simulink model "baseline_source"  (R2025a)
settings: Solver=daessc  StartTime=0.0  StopTime=25  MaxStep=5e-6  RelTol=1e-3
model workspace (MAT data in the model file):
  FocDiscrTime = 8.33333333333e-05
  Is_max = 420
  Ld = 0.00031
  Lq = 0.000305
  PolePairs = 11
  Psi = 0.1024
  Rs = 0.02
  VDC = 440
  compensate_dt = 0
  compensate_pwm = 0
  deltaLd = 0.2
  deltaLq = 0
  deltaPsi = 0
  deltaRs = 0
  mFW = 0.95
  mMaxCurrent = 0.99
  mMaxPWM = 0.99
  piBandwidth = 6000
libraries: fl_lib x18, nesl_utility x15, eeGeneralControl x9, mcbeeMathTransformLib x7, simulink x7, slpidlib x5, spsMeanLib x4, ee_lib x1, simulink_extras x1
(part 1 of 2)
settings Model: SimulationMode=rapid-accelerator  ExtModeTrigDuration=100  Creator=alexey  LastModifiedBy=alexey
settings SolverCC: ZeroCrossAlgorithm=Adaptive
settings OptimizationCC: DefaultParameterBehavior=Inlined  UseDivisionForNetSlopeComputation=on  GainParamInheritBuiltInType=on  UseFloatMulNetSlope=on  InlineInvariantSignals=on  ReuseModelBlockBuffer=off  EfficientFloat2IntCast=on  LifeSpan=1
settings DebuggingCC: MaskedZcDiagnostic=none  IgnoredZcDiagnostic=none
settings HardwareCC: ProdLongLongMode=on
settings SFSimCC: MATLABDynamicMemAlloc=off
settings RTWCC: GenerateReport=on  LaunchReport=on  GPUComputeCapability=3.5
settings CodeAppCC: ForceParamTrailComments=on
settings GRTTargetCC: RTWCAPISignals=on  RTWCAPIParams=on  CombineSignalStateStructs=on  MatFileLogging=off  SupportVariableSizeSignals=on

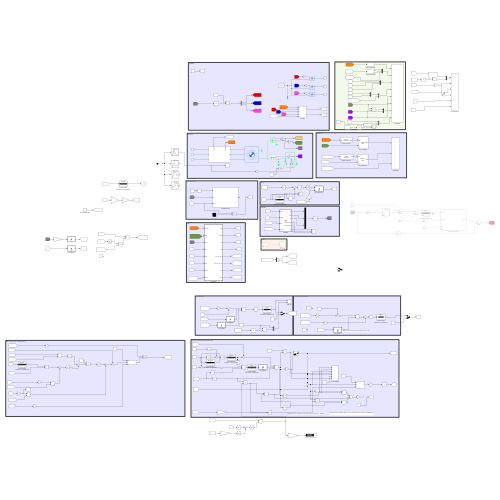
[thumbnail: Simulink's stored preview of the top-level diagram]
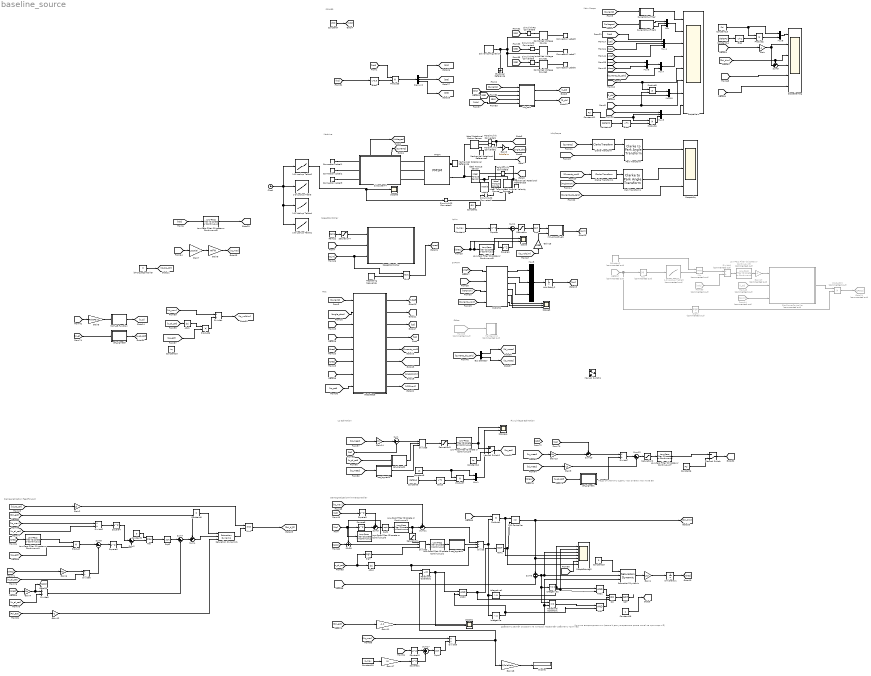
== system baseline_source ==
  note: Надо отключить оценку при омегах мех ниже 50
  note: Изучить вопрос динамики (роста U для ускоренного роста тока) на триммер и ff/
  note: Добавить расчёт скорости на которой перестаёт работать триммер
  note: Lq estimation
  note: Demagnetization FeedForward
  note: FluxLinkage Estimation
  note: Other
  note: SVPWM
  note: FOC
  note: IqLim
  note: DemagnetizationTrimmerController
  note: IdIqScope
  note: SpeedController
  note: Machine
  note: Main Scope
  note: POWER
  1-D Lookup Table : Lookup_n-D  NumberOfTableDimensions=1  BreakpointsForDimension1=[0 0.4 0.45 0.55 0.87 1 1.5 1.6 1.7]  Table=[0 308 308 104 104 120 120 220 220]  InternalRulePriority=Speed  RndMeth=Simplest
  1-D Lookup Table1 : Lookup_n-D  NumberOfTableDimensions=1  BreakpointsForDimension1=[0 0.2 0.4 4 4.2 8 8.2 9.0]  Table=[0 0 204 204 408 408 204 204]  InternalRulePriority=Speed  RndMeth=Simplest
  1-D Lookup Table2 : Lookup_n-D  NumberOfTableDimensions=1  BreakpointsForDimension1=[0 0.3 1 1.3 2 2.3 3 3.3 4 4.3 5 5.3 6 6.3 7 14 24 ]  Table=[0 104 104 208 208 312 312 416 416 520 520 624 624 738 738 156 21]  InternalRulePriority=Speed  RndMeth=Simplest
  1-D Lookup Table3 : Lookup_n-D  Commented=on  NumberOfTableDimensions=1  BreakpointsForDimension1=[0 550 600 1000 1925 2350 2400 2450]*0.1047  Table=[0 0 30000 48500 48500 22000 0 0]  InternalRulePriority=Speed  RndMeth=Simplest
  1-D Lookup Table4 : Lookup_n-D  NumberOfTableDimensions=1  BreakpointsForDimension1=[0 0.4 1.0 1.2 1.8]  Table=[0 408 408 204 204]  InternalRulePriority=Speed  RndMeth=Simplest
  AND : Logic  IconShape=distinctive  AllPortsSameDT=off  OutDataTypeStr=boolean
  AND1 : Logic  IconShape=distinctive  AllPortsSameDT=off  OutDataTypeStr=boolean
  AND2 : Logic  IconShape=distinctive  AllPortsSameDT=off  OutDataTypeStr=boolean
  Abs : Abs  Commented=on  SaturateOnIntegerOverflow=off
  Abs1 : Abs  SaturateOnIntegerOverflow=off
  Abs4 : Abs  SaturateOnIntegerOverflow=off
  Bias : Bias  Bias=1  SaturateOnIntegerOverflow=off
  Bias1 : Bias  Bias=1  SaturateOnIntegerOverflow=off
  Bias2 : Bias  Bias=-0.5  SaturateOnIntegerOverflow=off
  Bias3 : Bias  Bias=1  SaturateOnIntegerOverflow=off
  Bus Selector : BusSelector  OutputSignals=Id,Iq
  Clarke Transform : mcbeeMathTransformLib/Clarke Transform  VariantControl=Variant2  PowerInvariant=off  UseWithEmbedded=on  PhaseInput=Three inputs
      settings: LibrarySourceBlock=mcbcontrolslib/Clarke Transform
  Clarke Transform1 : mcbeeMathTransformLib/Clarke Transform  VariantControl=Variant2  PowerInvariant=off  UseWithEmbedded=on  PhaseInput=Three inputs
      settings: LibrarySourceBlock=mcbcontrolslib/Clarke Transform
  Clock : Clock
  Connection Label1 : ConnectionLabel  Label=A
  Connection Label2 : ConnectionLabel  Label=B
  Connection Label6 : ConnectionLabel  Label=C
  Connection Label7 : ConnectionLabel  Label=B
  Connection Label8 : ConnectionLabel  Label=A
  Connection Label9 : ConnectionLabel  Label=C
  Constant : Constant  Value=Is_max
  Constant1 : Constant  Value=-50
  Constant10 : Constant  Value=Lq
  Constant11 : Constant  Value=Psi
  Constant12 : Constant  Value=Lq  SampleTime=FocDiscrTime
  Constant13 : Constant  Value=Psi
  Constant14 : Constant  Value=deltaPsi
  Constant15 : Constant  Value=0
  Constant16 : Constant
  Constant18 : Constant  Value=Is_max
  Constant2 : Constant  Value=0
  Constant3 : Constant  Value=0
  Constant4 : Constant  Value=deltaPsi
  Constant5 : Constant  Commented=on  Value=48500
  Constant6 : Constant  Value=Psi  SampleTime=FocDiscrTime
  Constant7 : Constant  Value=VDC
  Constant8 : Constant  Value=Lq
  Constant9 : Constant  Value=deltaLq
  Controlled Voltage Source : fl_lib/Electrical/Electrical Sources/Controlled Voltage Source
  Controlled Voltage Source1 : fl_lib/Electrical/Electrical Sources/Controlled Voltage Source
  Controlled Voltage Source2 : fl_lib/Electrical/Electrical Sources/Controlled Voltage Source
  CurrentsMuxFilter : Subsystem
  CurrentsMuxFilter1 : Subsystem
  Demux2 : Demux  Outputs=3
  Display : Display
  Divide : Product  Inputs=*//
  Divide1 : Product  Commented=on  Inputs=*/
  Divide{2,4..7,9} (6 alike) : Product  Inputs=*/
  Divide3 : Product  Inputs=/**
  Divide8 : Product  Inputs=*//
  Electrical Reference : fl_lib/Electrical/Electrical Elements/Electrical Reference
  From38 : From  Commented=on  GotoTag=angle_mech
  From44 : From  Commented=on  GotoTag=IqLim
  From45 : From  Commented=on  GotoTag=I_dc
  From47 : From  Commented=on  GotoTag=speed
  From50 : From  Commented=on  GotoTag=Vdc
  Gain : Gain  Gain=-1
  Gain1 : Gain  Gain=1/Ld
  Gain10 : Gain  Commented=on  Gain=-1
  Gain11 : Gain  Gain=-1.2
  Gain12 : Gain  Gain=-1
  Gain{4,6,13..14} (4 alike) : Gain  Gain=Rs
  Gain15 : Gain  Gain=0.95
  Gain17 : Gain  Gain=Lq
  Gain18 : Gain  Gain=1/PolePairs
  Gain2 : Gain  Gain=Ld
  Gain3 : Gain  Gain=PolePairs
  Gain5 : Gain  Gain=PolePairs
  Gain7 : Gain  Gain=1/sqrt(3)
  Gain8 : Gain  Gain=mFW
  Gain9 : Gain  Gain=Ld
  GenPowerController : Subsystem  Commented=on
  Goto24 : Goto  Commented=on  GotoTag=IqReq1
  HallSensors : Subsystem  Commented=on
  Idc_calc : Subsystem
  Ideal Angular Velocity Source : fl_lib/Mechanical/Mechanical Sources/Ideal Angular Velocity Source
  Ideal Rotational Motion Sensor : fl_lib/Mechanical/Mechanical Sensors/Ideal Rotational Motion Sensor  reference=foundation.enum.MeasurementReference.difference  acceleration_port=false  velocity_port=true  position_port=true  wrap_angle=false  offset=0 rad
  Ideal Torque Sensor : fl_lib/Mechanical/Mechanical Sensors/Ideal Torque Sensor
  Ideal Torque Source : fl_lib/Mechanical/Mechanical Sources/Ideal Torque Source
  Inertia : fl_lib/Mechanical/Rotational Elements/Inertia  inertia=0.1 kg*m^2  num_ports=foundation.enum.numPorts2.one  w_specify=off  w_priority=High  w=0 rad/s  w_nominal_specify=off  w_nominal_value=1  w_nominal_unit=rad/s  t_specify=off  t_priority=None  t=0 N*m  t_nominal_specify=off  t_nominal_value=1  t_nominal_unit=N*m
  IsNegative : simulink/Logic and Bit Operations/Compare To Zero  relop=<  OutDataTypeStr=uint8
      settings: LibrarySourceBlock=|
      | simulink/Quick Insert/Logic and Bit
      | Operations/IsNegative
  IsNegative1 : simulink/Logic and Bit Operations/Compare To Zero  relop=>  OutDataTypeStr=uint8
      settings: LibrarySourceBlock=|
      | simulink/Quick Insert/Logic and Bit
      | Operations/IsNegative
  IsNegative2 : simulink/Logic and Bit Operations/Compare To Zero  relop=>=  OutDataTypeStr=uint8
      settings: LibrarySourceBlock=|
      | simulink/Quick Insert/Logic and Bit
      | Operations/IsNegative
  Low-Pass Filter (Discrete or Continuous)1 : eeGeneralControl/Low-Pass Filter (Discrete or Continuous)  K=1  T=FocDiscrTime*10  B=inf  A=-inf  init_option=Specify as parameter  x0=0  Ts=FocDiscrTime
  Low-Pass Filter (Discrete or Continuous)2 : eeGeneralControl/Low-Pass Filter (Discrete or Continuous)  K=1  T=FocDiscrTime*10  B=inf  A=-inf  init_option=Specify as parameter  x0=0  Ts=FocDiscrTime
  Low-Pass Filter (Discrete or Continuous)3 : eeGeneralControl/Low-Pass Filter (Discrete or Continuous)  Commented=on  K=1  T=FocDiscrTime*20  B=1.4*Psi  A=-inf  init_option=Specify as parameter  x0=Psi  Ts=FocDiscrTime
  Low-Pass Filter (Discrete or Continuous)4 : eeGeneralControl/Low-Pass Filter (Discrete or Continuous)  K=1  T=FocDiscrTime*10  B=inf  A=-inf  init_option=Inherited from block input  x0=0  Ts=FocDiscrTime
  Low-Pass Filter (Discrete or Continuous)5 : eeGeneralControl/Low-Pass Filter (Discrete or Continuous)  K=1  T=FocDiscrTime*20  B=inf  A=-inf  init_option=Specify as parameter  x0=VDC  Ts=FocDiscrTime
  Low-Pass Filter (Discrete or Continuous)6 : eeGeneralControl/Low-Pass Filter (Discrete or Continuous)  K=1  T=FocDiscrTime*10  B=inf  A=-inf  init_option=Specify as parameter  x0=0  Ts=FocDiscrTime
  Low-Pass Filter (Discrete or Continuous)7 : eeGeneralControl/Low-Pass Filter (Discrete or Continuous)  K=1  T=FocDiscrTime*20000  B=1.4*Psi  A=0.6*Psi  init_option=Specify as parameter  x0=Psi  Ts=FocDiscrTime
  Low-Pass Filter (Discrete or Continuous)8 : eeGeneralControl/Low-Pass Filter (Discrete or Continuous)  K=1  T=FocDiscrTime*100  B=inf  A=-inf  init_option=Specify as parameter  x0=0  Ts=FocDiscrTime
  Low-Pass Filter (Discrete or Continuous)9 : eeGeneralControl/Low-Pass Filter (Discrete or Continuous)  K=1  T=FocDiscrTime*200  B=inf  A=-inf  init_option=Specify as parameter  x0=Lq  Ts=FocDiscrTime
  MATLAB Function : MATLAB Function  TreatAsAtomicUnit=on
  Manual Switch : ManualSwitch  CurrentSetting=0
  Manual Switch1 : ManualSwitch
  Manual Switch2 : ManualSwitch  CurrentSetting=0
  Max : MinMax  Function=max  Inputs=2
  Mechanical Rotational Reference : fl_lib/Mechanical/Rotational Elements/Mechanical Rotational Reference
  Mechanical Rotational Reference2 : fl_lib/Mechanical/Rotational Elements/Mechanical Rotational Reference
  Mechanical Rotational Reference3 : fl_lib/Mechanical/Rotational Elements/Mechanical Rotational Reference
  Min : MinMax  Commented=on  Inputs=2
  Min1 : MinMax  Inputs=2
  Min3 : MinMax  Inputs=2
  Min_smooth_ab : MATLAB Function  TreatAsAtomicUnit=on
  Mux{,3..5} (4 alike) : Mux  Inputs=3
  Mux{1,6..8,10} (5 alike) : Mux  Inputs=2
  NOT : Logic  Operator=NOT  IconShape=distinctive  AllPortsSameDT=off  OutDataTypeStr=boolean
  NOT1 : Logic  Operator=NOT  IconShape=distinctive  AllPortsSameDT=off  OutDataTypeStr=boolean
  OR : Logic  Operator=OR  Inputs=3  IconShape=distinctive  AllPortsSameDT=off  OutDataTypeStr=boolean
  PID Controller : slpidlib/PID Controller  Controller=I  Form=Parallel  TimeDomain=Discrete-time  UseExternalTs=off  SampleTime=FocDiscrTime*1  IntegratorMethod=Forward Euler  FilterMethod=Forward Euler  ControllerParametersSource=internal  P=0  I=45  UseKiTs=off  D=0  UseExternalDerivativeSource=off  N=100  UseFilter=on  TunerSelectOption=Transfer Function Based (PID Tuner App)  InitialConditionSource=internal  InitialConditionForIntegrator=0  InitialConditionForFilter=0  DifferentiatorICPrevScaledInput=0  ExternalReset=either  TrackingMode=off  Kt=1  LimitOutput=on  SatLimitsSource=internal  UpperSaturationLimit=500*Ld  LowerSaturationLimit=-500*Ld  LinearizeAsGain=off  AntiWindupMode=clamping  Kb=1  LimitIntegrator=off  UpperIntegratorSaturationLimit=inf  LowerIntegratorSaturationLimit=-inf  RndMeth=Round  POutMin=[]  POutMax=[]  IOutMin=[]  IOutMax=[]  DOutMin=[]  DOutMax=[]  NOutMin=[]  NOutMax=[]  SumOutMin=[]  SumOutMax=[]  SaturationOutMin=[]  SaturationOutMax=[]  PParamMin=[]  PParamMax=[]  IParamMin=[]  IParamMax=[]  DParamMin=[]  DParamMax=[]  NParamMin=[]  NParamMax=[]  KbParamMin=[]  KbParamMax=[]  KtParamMin=[]  KtParamMax=[]  KbOutMin=[]  KbOutMax=[]  KtOutMin=[]  KtOutMax=[]  IntegratorOutMin=[]  IntegratorOutMax=[]  FilterOutMin=[]  FilterOutMax=[]  SumI1OutMin=[]  SumI1OutMax=[]  SumI2OutMin=[]  SumI2OutMax=[]  SumI3OutMin=[]  SumI3OutMax=[]  SumI4OutMin=[]  SumI4OutMax=[]  SumDOutMin=[]  SumDOutMax=[]  DifferentiatorOutMin=[]  DifferentiatorOutMax=[]  FilterDiffOutCoefMin=[]  FilterDiffOutCoefMax=[]  ReciprocalOutMin=[]  ReciprocalOutMax=[]  SumDenOutMin=[]  SumDenOutMax=[]  SumNumOutMin=[]  SumNumOutMax=[]  DivideOutMin=[]  DivideOutMax=[]  UdiffTsProdOutMin=[]  UdiffTsProdOutMax=[]  NTsProdOutMin=[]  NTsProdOutMax=[]  UintegralTsProdOutMin=[]  UintegralTsProdOutMax=[]  UngainTsProdOutMin=[]  UngainTsProdOutMax=[]  ClampingZeroOutDataTypeStr=Inherit: Inherit via back propagation  ClampingZeroOutMin=[]  ClampingZeroOutMax=[]  FilterDenConstantOutDataTypeStr=Inherit: Inherit via back propagation  FilterDenConstantOutMin=[]  FilterDenConstantOutMax=[]  PCopyOutDataTypeStr=Inherit: Inherit via back propagation  PCopyOutMin=[]  PCopyOutMax=[]  NCopyOutDataTypeStr=Inherit: Inherit via back propagation  NCopyOutMin=[]  NCopyOutMax=[]  IntegratorContinuousStateAttributes=''  IntegratorStateMustResolveToSignalObject=off  IntegratorRTWStateStorageClass=Auto  FilterContinuousStateAttributes=''  FilterStateMustResolveToSignalObject=off  FilterRTWStateStorageClass=Auto  ParallelPVariant=Disabled  IdealPVariant=Disabled  IVariant=InternalParameters  DVariant=Disabled  IntegratorVariant=Discrete  SatVariant=Enabled  AWVariant=DiscClampingParallel  PCopyVariant=Disabled  TRVariant=Disabled  FdbkBlocksVariant=Forward  IdealPFdbkVariant=Disabled  SatFdbkVariant=Disabled  DerivativeFilterVariant=Disabled  NVariant=Disabled  NCopyVariant=Disabled_SignalSpec  FilterICVariant=Disabled  IntegratorICVariant=InternalICs  ExternalResetVariant=ExternalReset  TRSumVariant=Passthrough  SumFdbkVariant=Disabled  SumVariant=Passthrough_I  TsampFilterVariant=InternalTs  TsampNgainVariant=Passthrough  TsampIntegralVariant=Disabled_SignalSpec  ExternalSaturationOutDataTypeStr=Inherit: Same as second input  DerivativeSourceVariant=Disabled  PreIntVariant=InternalPreInt
  PMSM : ee_lib/Electromechanical/Permanent Magnet/PMSM  port_option=ee.enum.threePhasePort.expanded  winding_type=ee.enum.electromech.statorconfiguration.wye  machine_param=ee.enum.pmsm.parameterization.constant  nPolePairs=PolePairs  pmflux_param=ee.enum.pmflux.fluxlinkage  pm_flux_linkage=Psi*(1+deltaPsi) Wb  torque_constant=0.074 N*m/A  back_emf_constant=0.06 V*s/rad  stator_param=ee.enum.statorparam.LdLqL0  Ld=Ld*(1+deltaLd) H  Lq=Lq*(1+deltaLq) H  idVec=[-200, 0, 200] A  iqVec=[-200, 0, 200] A  LdMatrix=0.0002 * ones(3, 3) H  LqMatrix=0.0002 * ones(3, 3) H  PmMatrix=0.1 * ones(3, 3) Wb  ktMatrix=0.18 * ones(3, 3) N*m/A  keMatrix=0.18 * ones(3, 3) V*s/rad  L0=1e-6 uH  Ls=0.0002 H  Lm=-0.00002 H  Ms=0.00002 H  Rs=Rs*(1+deltaRs) Ohm  zero_sequence=ee.enum.park.zerosequence.exclude  axes_param=ee.enum.rotorangle.daxis  loss_param=ee.enum.ironloss.none  losses_oc=[0, 0, 0] W  losses_sc=[0, 0, 0] W  f_losses=60 Hz  Isc_losses=95 A  J=0 kg*m^2  lam=0 N*m*s/rad  i_d_specify=on  i_d_priority=High  i_d=0 A  i_d_nominal_specify=off  i_d_nominal_value=1  i_d_nominal_unit=A  i_q_specify=on  i_q_priority=High  i_q=0 A  i_q_nominal_specify=off  i_q_nominal_value=1  i_q_nominal_unit=A  torque_specify=on  torque_priority=High  torque=0 N*m  torque_nominal_specify=off  torque_nominal_value=1  torque_nominal_unit=N*m  angular_velocity_specify=on  angular_velocity_priority=None  angular_velocity=7000 rpm  angular_velocity_nominal_specify=off  angular_velocity_nominal_value=1  angular_velocity_nominal_unit=rpm  angular_position_specify=on  angular_position_priority=High  angular_position=0 deg  angular_position_nominal_specify=off  angular_position_nominal_value=1  angular_position_nominal_unit=deg  alpha=3.93e-3 1/K  alpha_flux=-0.001 1/K  Tmeas=298.15 K  stator_thermal_mass=100 J/K  rotor_thermal_mass=200 J/K  Rm_percent_rotor=90  Rd_percent_rotor=30  temperatureA_specify=off  temperatureA_priority=High  temperatureA=25 degC  temperatureA_nominal_specify=off  temperatureA_nominal_value=1  temperatureA_nominal_unit=degC  temperatureB_specify=off  temperatureB_priority=High  temperatureB=25 degC  temperatureB_nominal_specify=off  temperatureB_nominal_value=1  temperatureB_nominal_unit=degC  temperatureC_specify=off  temperatureC_priority=High  temperatureC=25 degC  temperatureC_nominal_specify=off  temperatureC_nominal_value=1  temperatureC_nominal_unit=degC  temperatureR_specify=off  temperatureR_priority=High  temperatureR=25 degC  temperatureR_nominal_specify=off  temperatureR_nominal_value=1  temperatureR_nominal_unit=degC
      settings: InternalSimscapePortConfiguration="{\"Bottom\":[],\"Left\":[{\"id\":\"a\",\"label\":\"a\",\"type\":\"foundation.electrical.electrical\"},{\"id\":\"b\",\"label\":\"b\",\"type\":\"foundation.electrical.electrical\"},{\"id\":\"c\",\"label\":\"c\",\"type\":\"foundation.electrical.electrical\"}],\"Right\":[{\"id\":\"R\",\"label\":\"R\",\"type\":\"foundation.mechanical.rotational.rotational\"},{\"id\":\"C\",\"label\":\"C\",\"type\":\"foundation.mechanical.rotational.rotational\"}],\"Top\":[]}"
  PS-Simulink Converter1 : nesl_utility/PS-Simulink Converter  PhysicalDomain=network_engine_domain  SubClassName=ps_output  LeftPortType=input  RightPortType=output  PseudoPeriodic=off  Frequencies=[]  VectorFormat=inherit  Unit=inherit  AffineConversion=off
  PS-Simulink Converter2 : nesl_utility/PS-Simulink Converter  PhysicalDomain=network_engine_domain  SubClassName=ps_output  LeftPortType=input  RightPortType=output  PseudoPeriodic=off  Frequencies=[]  VectorFormat=inherit  Unit=inherit  AffineConversion=off
  PS-Simulink Converter3 : nesl_utility/PS-Simulink Converter  PhysicalDomain=network_engine_domain  SubClassName=ps_output  LeftPortType=input  RightPortType=output  PseudoPeriodic=off  Frequencies=[]  VectorFormat=inherit  Unit=inherit  AffineConversion=off
  Park Transform : mcbeeMathTransformLib/Clarke to Park Angle Transform  AxisAlignment=D-axis  UseWithEmbedded=on  PhaseInput=Three inputs  ThetaInput=Electrical position  AngleInput=Radians  N_points=1024
      settings: LibrarySourceBlock=mcbcontrolslib/Park Transform
  Park Transform1 : mcbeeMathTransformLib/Clarke to Park Angle Transform  AxisAlignment=D-axis  UseWithEmbedded=on  PhaseInput=Three inputs  ThetaInput=Electrical position  AngleInput=Radians  N_points=1024
      settings: LibrarySourceBlock=mcbcontrolslib/Park Transform
  Product{,1..7} (8 alike) : Product
  Product10 : Product  Commented=on
  Ramp2 : simulink/Sources/Ramp  slope=300/4e-3  start=1e-3  InitialOutput=0
  Relational Operator1 : RelationalOperator  Operator=<=  OutDataTypeStr=boolean  RndMeth=Simplest  InputSameDT=off
  Relational Operator2 : RelationalOperator  Operator=<=  OutDataTypeStr=boolean  RndMeth=Simplest  InputSameDT=off
  Repeating Sequence : simulink/Sources/Repeating Sequence  rep_seq_t=[0 0.2 0.5 0.7 1]  rep_seq_y=[Is_max -Is_max/10 -Is_max/10 Is_max Is_max]
  SVPWM1 : MATLAB Function  TreatAsAtomicUnit=on  SystemSampleTime=FocDiscrTime/2
  Saturation : Saturate  UpperLimit=inf  LowerLimit=0
  Saturation Dynamic : simulink/Discontinuities/Saturation Dynamic  OutMin=[]  OutMax=[]  OutDataTypeStr=Inherit: Same as second input  OutDataType=fixdt(1, 16)  OutScaling=2^-10  DoSatur=off
  Saturation Dynamic1 : simulink/Discontinuities/Saturation Dynamic  OutMin=[]  OutMax=[]  OutDataTypeStr=Inherit: Same as second input  OutDataType=fixdt(1, 16)  OutScaling=2^-10  DoSatur=off
  Saturation1 : Saturate  UpperLimit=inf  LowerLimit=1e-6
  Saturation2 : Saturate  UpperLimit=1.4*Psi  LowerLimit=0.6*Psi
  Saturation3 : Saturate  UpperLimit=1.4*Lq  LowerLimit=0.1*Lq
  Saturation4 : Saturate  UpperLimit=6000  LowerLimit=0
  Scope : Scope  NumInputPorts=2
      settings: ActiveDisplayYMinimum=-375.96970539923649  ActiveDisplayYMaximum=41.774411711026268  DataLoggingVariableName=ScopeData8
  Scope1 : Scope
      settings: ActiveDisplayYMinimum=-0.12499999999999997  ActiveDisplayYMaximum=1.125  DataLoggingVariableName=ScopeData7
  Scope3 : Scope  NumInputPorts=3
      settings: ActiveDisplayYMinimum=-1  ActiveDisplayYMaximum=1  DataLoggingVariableName=ScopeData12
  Scope6 : Scope
      settings: ActiveDisplayYMinimum=-68.247393749999986  ActiveDisplayYMaximum=614.22654375  DataLoggingVariableName=ScopeData15
  ScopeDemag : Scope  NumInputPorts=6
      settings: ActiveDisplayYMinimum=0.0023999999999999994  ActiveDisplayYMaximum=0.20240000000000002  DataLoggingVariableName=ScopeData14
  ScopeDemag2 : Scope  NumInputPorts=7
      settings: ActiveDisplayYMinimum=-0.12499999999999997  ActiveDisplayYMaximum=1.125  DataLoggingVariableName=ScopeData2
  ScopeIdIq : Scope  NumInputPorts=3
      settings: ActiveDisplayYMinimum=-510.04373604288077  ActiveDisplayYMaximum=523.61235955082839  DataLoggingDecimation=100  DataLoggingVariableName=ScopeData13
  ScopeLq : Scope  NumInputPorts=2
      settings: ActiveDisplayYMinimum=0.00022616516795357912  ActiveDisplayYMaximum=0.00033650286386801708
  ScopeMain : Scope  NumInputPorts=8
      settings: ActiveDisplayString=8  ActiveDisplayYMinimum=0.0023999999999999994  ActiveDisplayYMaximum=0.20240000000000002  DataLoggingVariableName=ScopeData9
  Sign : Signum
  Sign1 : Signum  Commented=on
  Simulink-PS Converter1 : nesl_utility/Simulink-PS Converter  PhysicalDomain=network_engine_domain  SubClassName=ps_input  LeftPortType=input  RightPortType=output  PseudoPeriodic=off  Frequencies=[]  NoiseDistribution=none  NoiseParameters=[]  Unit=1  AffineConversion=off  FilteringAndDerivatives=filter  SimscapeFilterOrder=1  InputFilterTimeConstant=1e-3  UdotUserProvided=0
  Simulink-PS Converter2 : nesl_utility/Simulink-PS Converter  PhysicalDomain=network_engine_domain  SubClassName=ps_input  LeftPortType=input  RightPortType=output  PseudoPeriodic=off  Frequencies=[]  NoiseDistribution=none  NoiseParameters=[]  Unit=1  AffineConversion=off  FilteringAndDerivatives=filter  SimscapeFilterOrder=1  InputFilterTimeConstant=1e-3  UdotUserProvided=0
  Simulink-PS Converter3 : nesl_utility/Simulink-PS Converter  PhysicalDomain=network_engine_domain  SubClassName=ps_input  LeftPortType=input  RightPortType=output  PseudoPeriodic=off  Frequencies=[]  NoiseDistribution=none  NoiseParameters=[]  Unit=1  AffineConversion=off  FilteringAndDerivatives=provide  SimscapeFilterOrder=1  InputFilterTimeConstant=0.001  UdotUserProvided=0
  Simulink-PS Converter4 : nesl_utility/Simulink-PS Converter  PhysicalDomain=network_engine_domain  SubClassName=ps_input  LeftPortType=input  RightPortType=output  PseudoPeriodic=off  Frequencies=[]  NoiseDistribution=none  NoiseParameters=[]  Unit=1  AffineConversion=off  FilteringAndDerivatives=provide  SimscapeFilterOrder=1  InputFilterTimeConstant=0.001  UdotUserProvided=0
  Simulink-PS Converter5 : nesl_utility/Simulink-PS Converter  PhysicalDomain=network_engine_domain  SubClassName=ps_input  LeftPortType=input  RightPortType=output  PseudoPeriodic=off  Frequencies=[]  NoiseDistribution=none  NoiseParameters=[]  Unit=1  AffineConversion=off  FilteringAndDerivatives=provide  SimscapeFilterOrder=1  InputFilterTimeConstant=0.001  UdotUserProvided=0
  Solver Configuration : nesl_utility/Solver Configuration  PhysicalDomain=network_engine_domain  SubClassName=solver  LeftPortType=input  RightPortType=generic  Tones=[]  Harmonics=[]  SimulateNoise=off  Profile=off  UseLocalSampling=off  EnableSwitchedLinearOptims=on  FrequencyDomain=off  UseCCode=off  RelTol=0.001  AbsTol=0.001  MinStep=1e-09  ToWorkspace=off  RevertToSquareIcSolve=off  NumHomotopyIterations=100  PhasorMode=off  PhasorModeNumHarmonics=1  ConsistencySolver=NEWTON_XTOL_AFTER_FTOL  IndexReductionMethod=DerivativeReplacement  DoDC=off  ResidualTolerance=1e-09  ConsistencyTolSource=GLOBAL  ConsistencyAbsTol=0.001  ConsistencyRelTol=0.001  ConsistencyTolFactor=0.001  UseLocalSolver=off  LocalSolverChoice=NE_BACKWARD_EULER_ADVANCER  ResolveIndetEquations=on  FunctionEvalNumThread=1  LocalSolverSampleTime=FocDiscrTime/10  DoFixedCost=off  MaxNonlinIter=3  MaxModeIter=2  ComputeImpulses=off  ImpulseIterations=2  LinearAlgebra=auto  LinearAlgebraNumThread=0  EquationFormulation=NE_TIME_EF  DelaysMemoryBudget=1024  AutomaticFiltering=on  FilteringTimeConstant=0.001  PartitionStorageMethod=AS_NEEDED  PartitionMemoryBudget=1024  PartitionMethod=ROBUST  MultibodyUseLocalSolver=off  MultibodyLocalSolverChoice=ODE1  MultibodyLocalSolverSampleTime=0.001
  SpeedController : Subsystem
  Sqrt{,1..2,4} (4 alike) : Sqrt
  Square{,1,3..5,8,10..11} (8 alike) : Math  Operator=square
  Subsystem4 : Subsystem
      settings: PortSchema="{\"entries\":[{\"content\":{\"sides\":[{\"content\":{},\"type\":\"ConnectorPlacement.EquallySpacedRectSide\",\"uuid\":\"18ff9a98-da5f-4d42-bf88-8b80acaefaab\"},{\"content\":{\"connectorIds\":[\"Out1\",\"Out2\"],\"side\":\"RIGHT\"},\"type\":\"ConnectorPlacement.EquallySpacedRectSide\",\"uuid\":\"2ae2e449-c022-4e43-8d74-e7903f555369\"},{\"content\":{\"connectorIds\":[\"LConn1\",\"LConn2\",\"LConn3\"],\"side\":\"TOP\"},\"type\":\"ConnectorPlacement.EquallySpacedRectSide\",\"uuid\":\"55b123c9-903d-428f-ba92-02a5913ccae5\"},{\"content\":{\"connectorIds\":[\"RConn1\",\"RConn2\",\"RConn3\"],\"side\":\"BOTTOM\"},\"type\":\"ConnectorPlacement.EquallySpacedRectSide\",\"uuid\":\"b028b0af-4fd3-4535-8d3b-f50dc0cabb29\"}]},\"type\":\"ConnectorPlacement.EquallySpacedConnector\",\"uuid\":\"08d0fd08-360e-4301-974e-a78b2c2bf0b9\"}],\"packageUris\":[\"http://schema.mathworks.com/mf0/Connector/R2020b\"],\"version\":\"1.0\"}"
  Sum{,1..2,7..8,12} (6 alike) : Sum  Inputs=|+-
  Sum10 : Sum  Inputs=+-|
  Sum11 : Sum  Inputs=+-|
  Sum17 : Sum  Inputs=|++
  Sum3 : Sum  Inputs=++|
  Sum4 : Sum  Inputs=-+|
  Sum5 : Sum  Inputs=-+|
  Sum6 : Sum
  Sum9 : Sum  Inputs=+-|
  Unit Delay1 : UnitDelay  SampleTime=FocDiscrTime/2  HasFrameUpgradeWarning=on
  Unit Delay2 : UnitDelay  SampleTime=FocDiscrTime/2  HasFrameUpgradeWarning=on
  VectorBase : Subsystem  TreatAsAtomicUnit=on  SystemSampleTime=FocDiscrTime
  idTorqueController : Constant  Value=0
  sat_signed1 : MATLAB Function  TreatAsAtomicUnit=on  SystemSampleTime=FocDiscrTime*10
  sat_signed2 : MATLAB Function  TreatAsAtomicUnit=on  SystemSampleTime=FocDiscrTime*10
  sat_signed3 : MATLAB Function  TreatAsAtomicUnit=on  SystemSampleTime=FocDiscrTime*10
  sat_signed4 : MATLAB Function  TreatAsAtomicUnit=on  SystemSampleTime=FocDiscrTime*10
  sat_signed5 : MATLAB Function  TreatAsAtomicUnit=on  SystemSampleTime=FocDiscrTime*10
  wires:
  [angle_elec] -> VectorBase/2(angle)
  Subsystem4/1(Voltages) -> [Voltages]
  CurrentsMuxFilter/1(Out2) -> ScopeMain/1
  [Currents] -> CurrentsMuxFilter/1(In1)
  Constant/1 -> Square/1
  PS-Simulink Converter3/1 -> [Torque]
  Mux/1 -> ScopeMain/2
  CurrentsMuxFilter1/1(Out1) -> Mux/1
  Saturation/1 -> Sqrt/1
  Sum1/1 -> Saturation/1
  [Torque] -> Product3/2, ScopeMain/6
  [speed] -> Product3/1, ScopeMain/5
  [Currents] -> VectorBase/1(currents)
  PS-Simulink Converter2/1 -> [speed]
  Square/1 -> Sum1/1
  Square1/1 -> Sum1/2
  [Vdc] -> Mux/3
  CurrentsMuxFilter1/2(Out2) -> Mux/2
  [Voltages] -> CurrentsMuxFilter1/1(In1)
  [Vdc] -> Low-Pass Filter (Discrete or Continuous)5/1
  Subsystem4/2(Currents) -> [Currents]
  [speed] -> VectorBase/3(speed)
  Gain3/1 -> [angle_elec]
  PS-Simulink Converter1/1 -> Gain3/1, [angle_mech]
  [Currents] -> Clarke Transform/1
  Clarke Transform/1 -> Park Transform/1
  [angle_elec] -> Park Transform/2
  Park Transform/1 -> ScopeIdIq/1
  [Currents_dq_calc] -> ScopeIdIq/3
  Ramp2/1 -> Saturation4/1
  [speed] -> SpeedController/2(In2)
  VectorBase/4(Vq) -> [Uq]
  [Idreq] -> VectorBase/5(Idreq)
  Saturation4/1 -> SpeedController/1(In1)
  VectorBase/5(Currents_work) -> [Currents_work]
  VectorBase/6(Currents_dq_calc) -> [Currents_dq_calc]
  Park Transform1/1 -> ScopeIdIq/2
  [AngleWork] -> Park Transform1/2
  Clarke Transform1/1 -> Park Transform1/1
  [Currents_work] -> Clarke Transform1/1
  VectorBase/3(Vd) -> [Ud]
  [Ud] -> Mux4/1
  [Uq] -> Mux4/2
  VectorBase/7(Ang) -> [AngleWork]
  Mux5/1 -> Unit Delay2/1
  Unit Delay2/1 -> [Kzi]
  VectorBase/2(vAngle) -> [vAngle]
  VectorBase/8(VDC) -> [VDCwork]
  VectorBase/1(vRef) -> [vRef]
  [vRef] -> SVPWM1/1(vRef)
  [Currents_work] -> SVPWM1/4(Currents)
  [vAngle] -> SVPWM1/2(vAngle)
  [VDCwork] -> SVPWM1/3(VDC)
  SVPWM1/1(Tat) -> Mux5/1
  SVPWM1/2(Tbt) -> Mux5/2
  SVPWM1/3(Tct) -> Mux5/3
  [IqLim] -> Min3/1, SpeedController/3(IqLim)
  Mux4/1 -> ScopeMain/3
  From38/1 -> HallSensors/1(In1)
  [Currents_dq_calc] -> Mux7/2
  [Idreq] -> Mux6/2
  [Iqreq] -> Mux6/1
  Mux6/1 -> Mux7/1
  Mux7/1 -> ScopeMain/4
  [vRef] -> Mux4/3
  Gain7/1 -> Gain8/1
  [Ud] -> Square3/1
  Square3/1 -> Sum3/1
  Constant1/1 -> Simulink-PS Converter2/1
  Clock/1 -> 1-D Lookup Table2/1, 1-D Lookup Table/1, 1-D Lookup Table1/1, 1-D Lookup Table4/1
  From44/1 -> GenPowerController/3(IqLim)
  From45/1 -> GenPowerController/2(Idc_meas)
  GenPowerController/1(IqReq) -> Product10/1
  From47/1 -> Sign1/1, Abs/1
  Low-Pass Filter (Discrete or Continuous)5/1 -> [Vdc_filt]
  Saturation Dynamic/1 -> Gain1/1
  [Uq] -> Low-Pass Filter (Discrete or Continuous)6/1, Square8/1
  Gain8/1 -> [Vs_max]
  Divide/1 -> IsNegative1/1, IsNegative/1, Product1/2
  Divide1/1 -> Low-Pass Filter (Discrete or Continuous)3/1
  From50/1 -> Divide1/2
  Low-Pass Filter (Discrete or Continuous)3/1 -> Gain10/1
  Demux2/3 -> [G5]
  Bias2/1 -> Product5/2
  Product5/1 -> Demux2/1
  Constant7/1 -> [Vdc]
  [G1] -> Simulink-PS Converter3/1
  Demux2/2 -> [G3]
  [Vdc] -> Product5/1
  Demux2/1 -> [G1]
  [Kzi] -> Bias2/1
  [G3] -> Simulink-PS Converter4/1
  [G5] -> Simulink-PS Converter5/1
  Abs/1 -> 1-D Lookup Table3/1
  1-D Lookup Table3/1 -> Min/2
  Constant5/1 -> Min/1
  Min/1 -> Divide1/1
  Product10/1 -> Goto24/1
  Sign1/1 -> Product10/2
  Gain10/1 -> GenPowerController/1(Idc_req)
  [Currents] -> Idc_calc/1(In1)
  [G1] -> Idc_calc/2(In2)
  [G3] -> Idc_calc/3(In3)
  [G5] -> Idc_calc/4(In4)
  Idc_calc/1(Out1) -> [I_dc]
  [Vdc] -> Idc_calc/5(In5)
  Idc_calc/2(Out2) -> [P_dc]
  [P_dc] -> Mux10/2
  [speed] -> Gain5/1
  Gain5/1 -> MATLAB Function/1(u)
  Constant2/1 -> Max/1
  [w_el_sat] -> Divide2/2
  Divide2/1 -> Square4/1
  Square4/1 -> Sum2/1
  Max/1 -> Sqrt2/1
  [Lq_est] -> Product/2
  Sum8/1 -> Square5/1
  Square5/1 -> Sum2/2
  Sum4/1 -> Saturation Dynamic1/2
  Saturation Dynamic1/1 -> Min1/2
  [Psi_est] -> Sum4/1
  Sqrt2/1 -> Sum7/1
  [Vs_max] -> Divide2/1
  [id_trq_ctrl] -> Gain2/1
  [Psi_d_ff] -> Sum6/2
  Low-Pass Filter (Discrete or Continuous)4/1 -> Product/1
  [Iqreq] -> Low-Pass Filter (Discrete or Continuous)4/1
  [Vs_max] -> Divide4/1
  [w_el_sat] -> Abs1/1
  [Lq_est] -> Product6/2
  Product6/1 -> Divide4/2
  Divide4/1 -> [Iq_voltLim]
  [Iq_voltLim] -> Gain15/1
  [Iqreq] -> VectorBase/6(Iqreq)
  Sqrt/1 -> Min_smooth_ab/1(a)
  Min_smooth_ab/1(y) -> [IqLim]
  [w_el_sat] -> Sign/1, Abs4/1
  [Vdc_filt] -> VectorBase/4(Vdc)
  [Vdc_filt] -> Gain7/1
  Square8/1 -> Sum3/2
  Sum3/1 -> Sqrt1/1
  Sqrt1/1 -> Low-Pass Filter (Discrete or Continuous)1/1
  Sum11/1 -> Divide/1
  MATLAB Function/1(y) -> [w_e]
  idTorqueController/1 -> [id_trq_ctrl]
  Saturation1/1 -> Divide3/1
  Gain11/1 -> Saturation Dynamic/3, Relational Operator1/2
  Relational Operator1/1 -> AND/1
  IsNegative/1 -> AND2/2, AND/2
  IsNegative2/1 -> ScopeDemag2/1, AND1/1
  IsNegative1/1 -> ScopeDemag2/2, AND1/2
  AND1/1 -> OR/1
  AND/1 -> OR/2
  OR/1 -> NOT/1
  [Psi_est] -> Mux3/1
  [Idreq] -> Square1/1, Scope/2, Low-Pass Filter (Discrete or Continuous)8/1
  NOT/1 -> ?
  [Psi_est] -> VectorBase/7(PsiEst)
  [freeze] -> Product1/1
  Product1/1 -> PID Controller/1, ScopeDemag2/4
  Constant11/1 -> Mux3/2, Product4/1
  Mux3/1 -> ScopeMain/8
  SVPWM1/5(overModulation) -> Scope3/1
  SVPWM1/6(viol) -> Scope3/2
  Sum6/1 -> ScopeDemag2/3, Saturation Dynamic/2, IsNegative2/1, Relational Operator1/1
  SVPWM1/4(vRefwork) -> Scope3/3
  [Psi_d_ff] -> Gain/1
  Constant14/1 -> Bias/1
  Bias/1 -> Product2/2
  Constant13/1 -> Mux8/1, Product2/1
  Gain/1 -> Sum5/2, ScopeDemag/2
  [Psi_trim] -> ScopeDemag/3, Sum5/1
  Sum5/1 -> ScopeDemag/4
  [Psi_est] -> ScopeDemag/5
  Product2/1 -> Mux8/2
  Sum2/1 -> Max/2
  [Iqreq] -> Gain4/1
  Gain4/1 -> [IqRs], Divide5/1
  [w_el_sat] -> Divide5/2
  Divide5/1 -> Sum7/2
  Sum7/1 -> Sum4/2
  [Idreq] -> Gain6/1
  Product/1 -> Sum8/1
  Gain6/1 -> Divide6/1
  [w_el_sat] -> Divide6/2
  Divide6/1 -> Sum8/2
  Mux8/1 -> ScopeDemag/1
  Min1/1 -> [Psi_d_ff]
  Divide3/1 -> Low-Pass Filter (Discrete or Continuous)2/1
  Sum9/1 -> Divide3/2  "E^?"
  sat_signed4/1(y) -> Divide/2
  Low-Pass Filter (Discrete or Continuous)2/1 -> sat_signed4/1(u)
  Constant15/1 -> Saturation Dynamic/1
  [Psi_est] -> Gain11/1
  1-D Lookup Table2/1 -> Simulink-PS Converter1/1, Scope6/1
  Product3/1 -> Mux10/1
  Mux10/1 -> ScopeMain/7
  [w_e] -> sat_signed5/1(u)
  sat_signed5/1(y) -> [w_el_sat]
  [IqRs] -> Sum9/2
  Gain2/1 -> Min1/1
  [Vs_max] -> Sum11/1
  Gain13/1 -> Sum10/2
  [Uq] -> Sum10/1
  [Id_meas] -> Gain9/1
  Gain9/1 -> Sum12/2
  [w_el_sat] -> sat_signed1/1(u)
  Sum10/1 -> Divide7/1  "E^?"
  Sum12/1 -> Saturation2/1
  Divide7/1 -> Sum12/1
  sat_signed1/1(y) -> Divide7/2
  [Psi_est] -> Gain12/1
  Constant3/1 -> Saturation Dynamic1/1
  Gain12/1 -> Saturation Dynamic1/3
  Bias1/1 -> Product4/2
  Constant4/1 -> Bias1/1
  Product4/1 -> Mux3/3
  Saturation2/1 -> Low-Pass Filter (Discrete or Continuous)7/1
  [Currents_dq_calc] -> Bus Selector/1
  Unit Delay1/1 -> [Idreq]
  Bus Selector/1 -> [Id_meas]  "<Id>"
  Bus Selector/2 -> [Iq_meas]  "<Iq>"
  [Iq_meas] -> Gain13/1
  [Id_meas] -> Gain14/1
  Gain14/1 -> Sum/1
  [Ud] -> Sum/2
  sat_signed2/1(y) -> Divide8/2
  [w_el_sat] -> sat_signed2/1(u)
  Sum/1 -> Divide8/1
  [Iq_meas] -> sat_signed3/1(u)
  Divide8/1 -> Saturation3/1
  Low-Pass Filter (Discrete or Continuous)9/1 -> Manual Switch2/1, ScopeLq/1
  sat_signed3/1(y) -> Divide8/3
  Saturation3/1 -> Low-Pass Filter (Discrete or Continuous)9/1
  [Lq_est] -> VectorBase/8(LqEst)
  [freeze] -> ScopeDemag/6
  Constant9/1 -> Bias3/1
  Bias3/1 -> Product7/2
  Constant8/1 -> Mux1/1, Product7/1
  Product7/1 -> Mux1/2
  Mux1/1 -> ScopeLq/2
  Gain1/1 -> Unit Delay1/1
  Abs4/1 -> Relational Operator2/1, Divide/3
  Gain18/1 -> Display/1
  Relational Operator2/1 -> Scope1/1, AND2/1
  NOT1/1 -> ScopeDemag2/7, PID Controller/2
  Constant18/1 -> Gain17/1
  Divide9/1 -> Gain18/1, Relational Operator2/2
  [Vs_max] -> Divide9/1
  [Psi_est] -> Square10/1
  Square10/1 -> Sum17/1
  Square11/1 -> Sum17/2
  Gain17/1 -> Square11/1
  Sum17/1 -> Sqrt4/1
  Sqrt4/1 -> Divide9/2
  AND2/1 -> NOT1/1, OR/3
  Min3/1 -> [Iqreq]
  Repeating Sequence/1 -> Min3/2
  [freeze] -> ScopeDemag2/6
  PID Controller/1 -> Sum6/1, ScopeDemag2/5, [Psi_trim]
  Abs1/1 -> Product6/1
  Sign/1 -> Divide3/3
  Low-Pass Filter (Discrete or Continuous)8/1 -> Scope/1
  Manual Switch/1 -> [Psi_est]
  Low-Pass Filter (Discrete or Continuous)7/1 -> Manual Switch/1
  Constant6/1 -> Manual Switch/2
  Manual Switch2/1 -> [Lq_est]
  Constant12/1 -> Manual Switch2/2
  Gain15/1 -> Min_smooth_ab/2(b)
  Low-Pass Filter (Discrete or Continuous)1/1 -> Sum11/2, Saturation1/1
  Low-Pass Filter (Discrete or Continuous)6/1 -> Sum9/1
  Constant16/1 -> [freeze]
  connections:
  Ideal Torque Sensor/LConn1 -- PMSM/RConn1 -- Ideal Rotational Motion Sensor/LConn1
  Simulink-PS Converter1/RConn1 -- Ideal Angular Velocity Source/RConn1
  Mechanical Rotational Reference3/LConn1 -- Ideal Torque Source/LConn1 -- Ideal Angular Velocity Source/RConn2 -- Ideal Torque Source/RConn2
  PMSM/LConn3 -- Subsystem4/RConn3
  Connection Label2/LConn1 -- Subsystem4/LConn2
  PS-Simulink Converter3/LConn1 -- Ideal Torque Sensor/RConn2
  PS-Simulink Converter1/LConn1 -- Ideal Rotational Motion Sensor/RConn3
  PMSM/LConn2 -- Subsystem4/RConn2
  Connection Label1/LConn1 -- Subsystem4/LConn3
  PMSM/RConn2 -- Mechanical Rotational Reference/LConn1
  PS-Simulink Converter2/LConn1 -- Ideal Rotational Motion Sensor/RConn2
  Connection Label9/LConn1 -- Subsystem4/LConn1
  PMSM/LConn1 -- Subsystem4/RConn1
  Ideal Rotational Motion Sensor/RConn1 -- Mechanical Rotational Reference2/LConn1
  Ideal Torque Sensor/RConn1 -- Ideal Angular Velocity Source/LConn1 -- Inertia/LConn1
  Simulink-PS Converter2/RConn1 -- Ideal Torque Source/RConn1
  Controlled Voltage Source1/RConn2 -- Controlled Voltage Source/RConn2 -- Solver Configuration/RConn1 -- Electrical Reference/LConn1 -- Controlled Voltage Source2/RConn2
  Simulink-PS Converter5/RConn1 -- Controlled Voltage Source2/RConn1
  Simulink-PS Converter3/RConn1 -- Controlled Voltage Source/RConn1
  Simulink-PS Converter4/RConn1 -- Controlled Voltage Source1/RConn1
  Connection Label7/LConn1 -- Controlled Voltage Source1/LConn1
  Connection Label6/LConn1 -- Controlled Voltage Source2/LConn1
  Connection Label8/LConn1 -- Controlled Voltage Source/LConn1

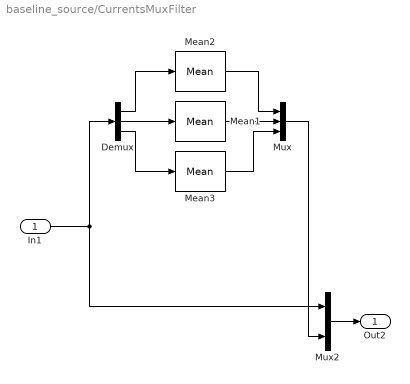
== system baseline_source/CurrentsMuxFilter ==
  In1 : Inport
  Demux : Demux  Outputs=3
  Mean1 : spsMeanLib/Mean  Freq=20000  Vinit=0  Ts=0
  Mean2 : spsMeanLib/Mean  Freq=20000  Vinit=0  Ts=0
  Mean3 : spsMeanLib/Mean  Freq=20000  Vinit=0  Ts=0
  Mux : Mux  Inputs=3
  Mux2 : Mux  Inputs=2
  Out2 : Outport
  wires:
  Mean3/1 -> Mux/3
  Mean1/1 -> Mux/2
  Mean2/1 -> Mux/1
  Demux/3 -> Mean3/1
  Demux/2 -> Mean1/1
  Demux/1 -> Mean2/1
  Mux2/1 -> Out2/1
  In1/1 -> Mux2/1, Demux/1
  Mux/1 -> Mux2/2

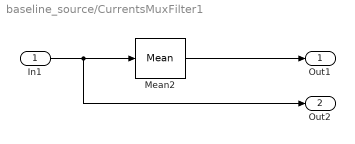
== system baseline_source/CurrentsMuxFilter1 ==
  In1 : Inport
  Mean2 : spsMeanLib/Mean  Freq=20000  Vinit=0  Ts=0
  Out1 : Outport
  Out2 : Outport  Port=2
  wires:
  In1/1 -> Mean2/1, Out2/1
  Mean2/1 -> Out1/1

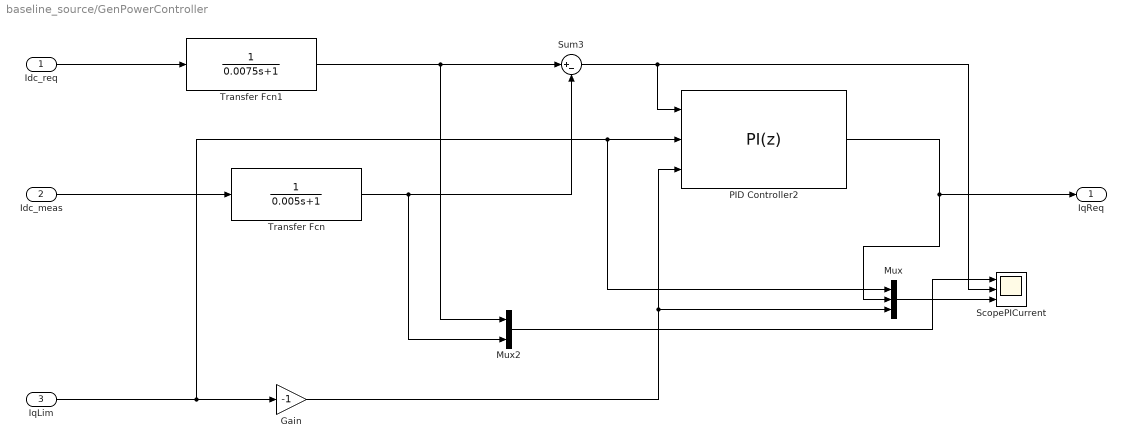
== system baseline_source/GenPowerController ==
  Idc_req : Inport
  Idc_meas : Inport  Port=2
  IqLim : Inport  Port=3
  Gain : Gain  Gain=-1
  Mux : Mux  Inputs=3
  Mux2 : Mux  Inputs=2
  PID Controller2 : slpidlib/PID Controller  Controller=PI  Form=Parallel  TimeDomain=Discrete-time  UseExternalTs=off  SampleTime=FocDiscrTime  IntegratorMethod=Forward Euler  FilterMethod=Forward Euler  ControllerParametersSource=internal  P=5  I=450  UseKiTs=off  D=0  UseExternalDerivativeSource=off  N=100  UseFilter=on  TunerSelectOption=Transfer Function Based (PID Tuner App)  InitialConditionSource=internal  InitialConditionForIntegrator=0  InitialConditionForFilter=0  DifferentiatorICPrevScaledInput=0  ExternalReset=none  TrackingMode=off  Kt=1  LimitOutput=on  SatLimitsSource=external  UpperSaturationLimit=350  LowerSaturationLimit=-3  LinearizeAsGain=on  AntiWindupMode=clamping  Kb=1  LimitIntegrator=off  UpperIntegratorSaturationLimit=inf  LowerIntegratorSaturationLimit=-inf  POutMin=[]  POutMax=[]  IOutMin=[]  IOutMax=[]  DOutMin=[]  DOutMax=[]  NOutMin=[]  NOutMax=[]  SumOutMin=[]  SumOutMax=[]  SaturationOutMin=[]  SaturationOutMax=[]  PParamMin=[]  PParamMax=[]  IParamMin=[]  IParamMax=[]  DParamMin=[]  DParamMax=[]  NParamMin=[]  NParamMax=[]  KbParamMin=[]  KbParamMax=[]  KtParamMin=[]  KtParamMax=[]  KbOutMin=[]  KbOutMax=[]  KtOutMin=[]  KtOutMax=[]  IntegratorOutMin=[]  IntegratorOutMax=[]  FilterOutMin=[]  FilterOutMax=[]  SumI1OutMin=[]  SumI1OutMax=[]  SumI2OutMin=[]  SumI2OutMax=[]  SumI3OutMin=[]  SumI3OutMax=[]  SumI4OutMin=[]  SumI4OutMax=[]  SumDOutMin=[]  SumDOutMax=[]  DifferentiatorOutMin=[]  DifferentiatorOutMax=[]  FilterDiffOutCoefMin=[]  FilterDiffOutCoefMax=[]  ReciprocalOutMin=[]  ReciprocalOutMax=[]  SumDenOutMin=[]  SumDenOutMax=[]  SumNumOutMin=[]  SumNumOutMax=[]  DivideOutMin=[]  DivideOutMax=[]  UdiffTsProdOutMin=[]  UdiffTsProdOutMax=[]  NTsProdOutMin=[]  NTsProdOutMax=[]  UintegralTsProdOutMin=[]  UintegralTsProdOutMax=[]  UngainTsProdOutMin=[]  UngainTsProdOutMax=[]  ClampingZeroOutDataTypeStr=Inherit: Inherit via back propagation  ClampingZeroOutMin=[]  ClampingZeroOutMax=[]  FilterDenConstantOutDataTypeStr=Inherit: Inherit via back propagation  FilterDenConstantOutMin=[]  FilterDenConstantOutMax=[]  PCopyOutDataTypeStr=Inherit: Inherit via back propagation  PCopyOutMin=[]  PCopyOutMax=[]  NCopyOutDataTypeStr=Inherit: Inherit via back propagation  NCopyOutMin=[]  NCopyOutMax=[]  IntegratorContinuousStateAttributes=''  IntegratorStateMustResolveToSignalObject=off  IntegratorRTWStateStorageClass=Auto  FilterContinuousStateAttributes=''  FilterStateMustResolveToSignalObject=off  FilterRTWStateStorageClass=Auto  ParallelPVariant=InternalParameters  IdealPVariant=Disabled  IVariant=InternalParameters  DVariant=Disabled  IntegratorVariant=Discrete  SatVariant=External  AWVariant=DiscClampingParallel  PCopyVariant=Disabled  TRVariant=Disabled  FdbkBlocksVariant=Forward  IdealPFdbkVariant=Disabled  SatFdbkVariant=Disabled  DerivativeFilterVariant=Disabled  NVariant=Disabled  NCopyVariant=Disabled_SignalSpec  FilterICVariant=Disabled  IntegratorICVariant=InternalICs  ExternalResetVariant=Disabled  TRSumVariant=Passthrough  SumFdbkVariant=Disabled  SumVariant=Sum_PI  TsampFilterVariant=InternalTs  TsampNgainVariant=Passthrough  TsampIntegralVariant=Disabled_SignalSpec  ExternalSaturationOutDataTypeStr=Inherit: Same as second input  DerivativeSourceVariant=Disabled  PreIntVariant=InternalPreInt
  ScopePICurrent : Scope  NumInputPorts=3
      settings: ActiveDisplayYMinimum=-166.72089000317976  ActiveDisplayYMaximum=287.98832865297436  DataLoggingVariableName=ScopeData10
  Sum3 : Sum  Inputs=|+-
  Transfer Fcn : TransferFcn  Denominator=[0.005 1]
  Transfer Fcn1 : TransferFcn  Denominator=[0.0075 1]
  IqReq : Outport
  wires:
  Idc_req/1 -> Transfer Fcn1/1
  Transfer Fcn/1 -> Sum3/2, Mux2/2
  Sum3/1 -> PID Controller2/1, ScopePICurrent/2
  Mux2/1 -> ScopePICurrent/1
  Idc_meas/1 -> Transfer Fcn/1
  PID Controller2/1 -> Mux/2, IqReq/1
  IqLim/1 -> PID Controller2/2, Mux/1, Gain/1
  Gain/1 -> PID Controller2/3, Mux/3
  Transfer Fcn1/1 -> Mux2/1, Sum3/1
  Mux/1 -> ScopePICurrent/3

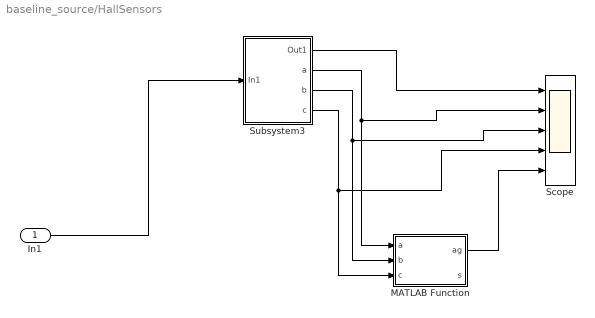
== system baseline_source/HallSensors ==
  In1 : Inport
  MATLAB Function : MATLAB Function  TreatAsAtomicUnit=on  SystemSampleTime=1/(FocDiscrTime/2)
  Scope : Scope  NumInputPorts=5
      settings: ActiveDisplayYMinimum=-0.7854  ActiveDisplayYMaximum=7.06858  DataLoggingVariableName=ScopeData3
  Subsystem3 : Subsystem
  wires:
  In1/1 -> Subsystem3/1(In1)
  Subsystem3/3(b) -> MATLAB Function/2(b), Scope/3
  MATLAB Function/1(ag) -> Scope/5
  Subsystem3/2("a ") -> MATLAB Function/1(a), Scope/2
  Subsystem3/4(c) -> MATLAB Function/3(c), Scope/4
  Subsystem3/1(Out1) -> Scope/1

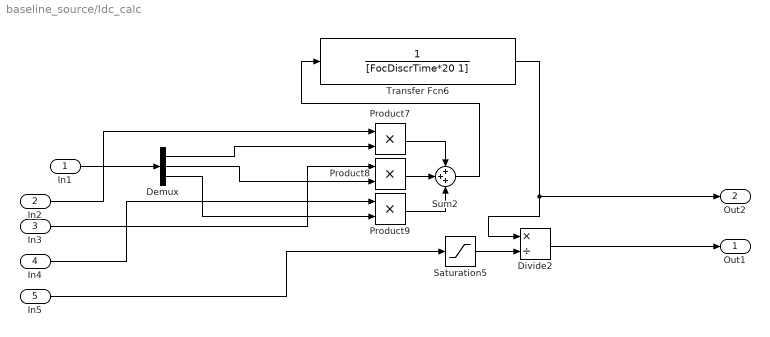
== system baseline_source/Idc_calc ==
  In1 : Inport
  In2 : Inport  Port=2
  In3 : Inport  Port=3
  In4 : Inport  Port=4
  In5 : Inport  Port=5
  Demux : Demux  Outputs=3
  Divide2 : Product  Inputs=*/
  Product7 : Product
  Product8 : Product
  Product9 : Product
  Saturation5 : Saturate  UpperLimit=inf  LowerLimit=1e-5
  Sum2 : Sum  Inputs=+++
  Transfer Fcn6 : TransferFcn  Denominator=[FocDiscrTime*20 1]
  Out1 : Outport
  Out2 : Outport  Port=2
  wires:
  In3/1 -> Product8/1
  Product9/1 -> Sum2/3
  Divide2/1 -> Out1/1
  In1/1 -> Demux/1
  Product7/1 -> Sum2/1
  Product8/1 -> Sum2/2
  In4/1 -> Product9/1
  Demux/1 -> Product7/2
  In5/1 -> Saturation5/1
  Sum2/1 -> Transfer Fcn6/1
  In2/1 -> Product7/1
  Transfer Fcn6/1 -> Divide2/1, Out2/1
  Demux/3 -> Product9/2
  Demux/2 -> Product8/2
  Saturation5/1 -> Divide2/2

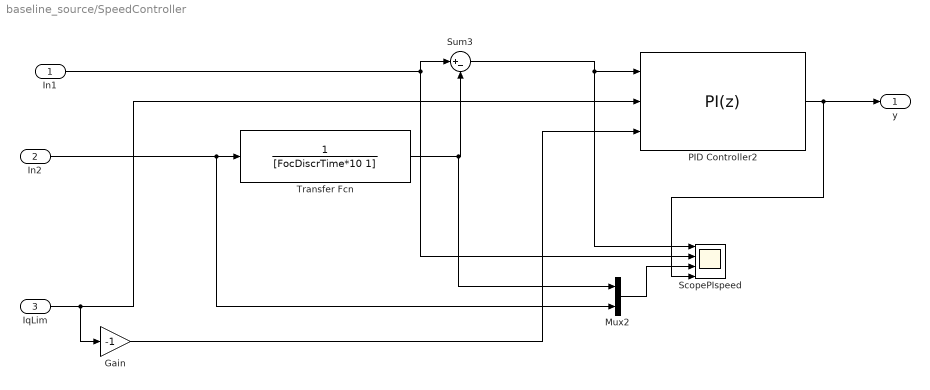
== system baseline_source/SpeedController ==
  In1 : Inport
  In2 : Inport  Port=2
  IqLim : Inport  Port=3
  Gain : Gain  Gain=-1
  Mux2 : Mux  Inputs=2
  PID Controller2 : slpidlib/PID Controller  Controller=PI  Form=Parallel  TimeDomain=Discrete-time  UseExternalTs=off  SampleTime=FocDiscrTime  IntegratorMethod=Forward Euler  FilterMethod=Forward Euler  ControllerParametersSource=internal  P=5  I=1  UseKiTs=off  D=0  UseExternalDerivativeSource=off  N=100  UseFilter=on  TunerSelectOption=Transfer Function Based (PID Tuner App)  InitialConditionSource=internal  InitialConditionForIntegrator=0  InitialConditionForFilter=0  DifferentiatorICPrevScaledInput=0  ExternalReset=none  TrackingMode=off  Kt=1  LimitOutput=on  SatLimitsSource=external  UpperSaturationLimit=350  LowerSaturationLimit=-3  LinearizeAsGain=on  AntiWindupMode=clamping  Kb=1  LimitIntegrator=off  UpperIntegratorSaturationLimit=inf  LowerIntegratorSaturationLimit=-inf  POutMin=[]  POutMax=[]  IOutMin=[]  IOutMax=[]  DOutMin=[]  DOutMax=[]  NOutMin=[]  NOutMax=[]  SumOutMin=[]  SumOutMax=[]  SaturationOutMin=[]  SaturationOutMax=[]  PParamMin=[]  PParamMax=[]  IParamMin=[]  IParamMax=[]  DParamMin=[]  DParamMax=[]  NParamMin=[]  NParamMax=[]  KbParamMin=[]  KbParamMax=[]  KtParamMin=[]  KtParamMax=[]  KbOutMin=[]  KbOutMax=[]  KtOutMin=[]  KtOutMax=[]  IntegratorOutMin=[]  IntegratorOutMax=[]  FilterOutMin=[]  FilterOutMax=[]  SumI1OutMin=[]  SumI1OutMax=[]  SumI2OutMin=[]  SumI2OutMax=[]  SumI3OutMin=[]  SumI3OutMax=[]  SumI4OutMin=[]  SumI4OutMax=[]  SumDOutMin=[]  SumDOutMax=[]  DifferentiatorOutMin=[]  DifferentiatorOutMax=[]  FilterDiffOutCoefMin=[]  FilterDiffOutCoefMax=[]  ReciprocalOutMin=[]  ReciprocalOutMax=[]  SumDenOutMin=[]  SumDenOutMax=[]  SumNumOutMin=[]  SumNumOutMax=[]  DivideOutMin=[]  DivideOutMax=[]  UdiffTsProdOutMin=[]  UdiffTsProdOutMax=[]  NTsProdOutMin=[]  NTsProdOutMax=[]  UintegralTsProdOutMin=[]  UintegralTsProdOutMax=[]  UngainTsProdOutMin=[]  UngainTsProdOutMax=[]  ClampingZeroOutDataTypeStr=Inherit: Inherit via back propagation  ClampingZeroOutMin=[]  ClampingZeroOutMax=[]  FilterDenConstantOutDataTypeStr=Inherit: Inherit via back propagation  FilterDenConstantOutMin=[]  FilterDenConstantOutMax=[]  PCopyOutDataTypeStr=Inherit: Inherit via back propagation  PCopyOutMin=[]  PCopyOutMax=[]  NCopyOutDataTypeStr=Inherit: Inherit via back propagation  NCopyOutMin=[]  NCopyOutMax=[]  IntegratorContinuousStateAttributes=''  IntegratorStateMustResolveToSignalObject=off  IntegratorRTWStateStorageClass=Auto  FilterContinuousStateAttributes=''  FilterStateMustResolveToSignalObject=off  FilterRTWStateStorageClass=Auto  ParallelPVariant=InternalParameters  IdealPVariant=Disabled  IVariant=InternalParameters  DVariant=Disabled  IntegratorVariant=Discrete  SatVariant=External  AWVariant=DiscClampingParallel  PCopyVariant=Disabled  TRVariant=Disabled  FdbkBlocksVariant=Forward  IdealPFdbkVariant=Disabled  SatFdbkVariant=Disabled  DerivativeFilterVariant=Disabled  NVariant=Disabled  NCopyVariant=Disabled_SignalSpec  FilterICVariant=Disabled  IntegratorICVariant=InternalICs  ExternalResetVariant=Disabled  TRSumVariant=Passthrough  SumFdbkVariant=Disabled  SumVariant=Sum_PI  TsampFilterVariant=InternalTs  TsampNgainVariant=Passthrough  TsampIntegralVariant=Disabled_SignalSpec  ExternalSaturationOutDataTypeStr=Inherit: Same as second input  DerivativeSourceVariant=Disabled  PreIntVariant=InternalPreInt
  ScopePIspeed : Scope  NumInputPorts=4
      settings: ActiveDisplayYMinimum=-746.615895073923  ActiveDisplayYMaximum=6719.1301611810532  DataLoggingVariableName=ScopeData10
  Sum3 : Sum  Inputs=|+-
  Transfer Fcn : TransferFcn  Denominator=[FocDiscrTime*10 1]
  y : Outport
  wires:
  Mux2/1 -> ScopePIspeed/3
  In2/1 -> Mux2/2, Transfer Fcn/1
  PID Controller2/1 -> y/1, ScopePIspeed/4
  Sum3/1 -> ScopePIspeed/1, PID Controller2/1
  Transfer Fcn/1 -> Mux2/1, Sum3/2
  In1/1 -> Sum3/1, ScopePIspeed/2
  IqLim/1 -> Gain/1, PID Controller2/2
  Gain/1 -> PID Controller2/3

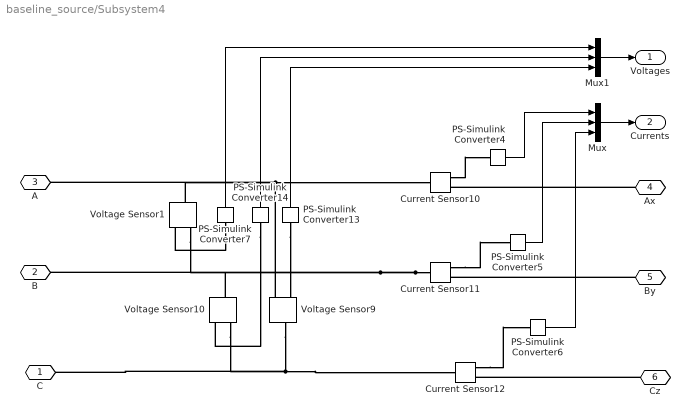
== system baseline_source/Subsystem4 ==
  Current Sensor10 : fl_lib/Electrical/Electrical Sensors/Current Sensor
  Current Sensor11 : fl_lib/Electrical/Electrical Sensors/Current Sensor
  Current Sensor12 : fl_lib/Electrical/Electrical Sensors/Current Sensor
  Mux : Mux  Inputs=3
  Mux1 : Mux  Inputs=3
  PS-Simulink Converter{4..7,13..14} (6 alike) : nesl_utility/PS-Simulink Converter  PhysicalDomain=network_engine_domain  SubClassName=ps_output  LeftPortType=input  RightPortType=output  PseudoPeriodic=off  Frequencies=[]  VectorFormat=inherit  Unit=inherit  AffineConversion=off
  Voltage Sensor1 : fl_lib/Electrical/Electrical Sensors/Voltage Sensor
  Voltage Sensor10 : fl_lib/Electrical/Electrical Sensors/Voltage Sensor
  Voltage Sensor9 : fl_lib/Electrical/Electrical Sensors/Voltage Sensor
  C : PMIOPort  Side=Left
  B : PMIOPort  Port=2  Side=Left
  A : PMIOPort  Port=3  Side=Left
  Ax : PMIOPort  Port=4  Side=Right
  By : PMIOPort  Port=5  Side=Right
  Cz : PMIOPort  Port=6  Side=Right
  Voltages : Outport
  Currents : Outport  Port=2
  wires:
  Mux1/1 -> Voltages/1
  Mux/1 -> Currents/1
  PS-Simulink Converter7/1 -> Mux1/1
  PS-Simulink Converter14/1 -> Mux1/2
  PS-Simulink Converter4/1 -> Mux/1
  PS-Simulink Converter13/1 -> Mux1/3
  PS-Simulink Converter6/1 -> Mux/3
  PS-Simulink Converter5/1 -> Mux/2
  connections:
  By/RConn1 -- Current Sensor11/RConn2
  PS-Simulink Converter7/LConn1 -- Voltage Sensor1/RConn1
  PS-Simulink Converter14/LConn1 -- Voltage Sensor10/RConn1
  Current Sensor11/LConn1 -- Voltage Sensor1/RConn2 -- B/RConn1 -- Voltage Sensor10/LConn1
  Current Sensor12/RConn1 -- PS-Simulink Converter6/LConn1
  Voltage Sensor9/RConn2 -- Current Sensor10/LConn1 -- A/RConn1 -- Voltage Sensor1/LConn1
  Voltage Sensor9/LConn1 -- Current Sensor12/LConn1 -- C/RConn1 -- Voltage Sensor10/RConn2
  Current Sensor11/RConn1 -- PS-Simulink Converter5/LConn1
  Cz/RConn1 -- Current Sensor12/RConn2
  Current Sensor10/RConn1 -- PS-Simulink Converter4/LConn1
  PS-Simulink Converter13/LConn1 -- Voltage Sensor9/RConn1
  Ax/RConn1 -- Current Sensor10/RConn2
